simulink model "NGW_mech_only"  (R2023b)
settings: Solver=ode15s  StartTime=0  StopTime=0.3  MaxStep=2e-4  RelTol=1e-7  AbsTol=1e-9
InitFcn:
  | NGW_init
values from neighbouring files (symbols this model uses):
  cL = 0    [NGW_init.m]    (also in NGW_test.m = 0.5)
  Te_cmd = 2.0    (= 2)    [NGW_init.m]
undefined symbols (not defined in the file or in its folder): NGW_params
settings Model: Creator=Administrator  LastModifiedBy=Administrator

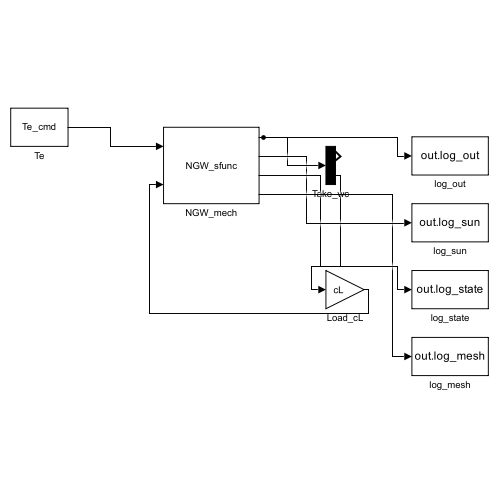
[thumbnail: Simulink's stored preview of the top-level diagram]
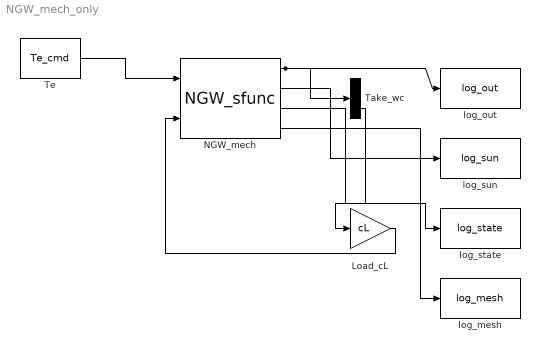
== system NGW_mech_only ==
  Load_cL : Gain  Gain=cL
  NGW_mech : M-S-Function  FunctionName=NGW_sfunc  Parameters=NGW_params()
  Take_wc : Demux  Outputs=2
  Te : Constant  Value=Te_cmd
  log_mesh : ToWorkspace  VariableName=log_mesh  SaveFormat=Timeseries  SampleTime=-1
  log_out : ToWorkspace  VariableName=log_out  SaveFormat=Timeseries  SampleTime=-1
  log_state : ToWorkspace  VariableName=log_state  SaveFormat=Timeseries  SampleTime=-1
  log_sun : ToWorkspace  VariableName=log_sun  SaveFormat=Timeseries  SampleTime=-1
  wires:
  Te/1 -> NGW_mech/1
  NGW_mech/1 -> Take_wc/1, log_out/1
  Take_wc/2 -> Load_cL/1
  Load_cL/1 -> NGW_mech/2
  NGW_mech/2 -> log_sun/1
  NGW_mech/3 -> log_state/1
  NGW_mech/4 -> log_mesh/1
